simulink model "rfsoc4x2_ospfb_128"  (R2021a)
settings: Solver=VariableStepAuto  StartTime=0.0  StopTime=2048  RelTol=1e-3
undefined symbols (not defined in the file): pfb_coeff_gen_calc
libraries: xbsIndex_r4 x37092, casper_library_delays x737, casper_library_misc x68, xps_library x1
(part 117 of 339)

== system rfsoc4x2_ospfb_128/pfb_fir_real8/pol1_in2_coeffs ==
  din : Inport
  sync : Inport  Port=2
  Concat : xbsIndex_r4/Concat  num_inputs=4  dbl_ovrd=off  block_type=concat
      settings: block_version=9.1.01
  Counter : xbsIndex_r4/Counter  cnt_type=Free Running  cnt_to=Inf  operation=Up  start_count=0  cnt_by_val=1  arith_type=Unsigned  n_bits=4  bin_pt=0  load_pin=off  rst=on  en=off  explicit_period=on  period=1  use_behavioral_HDL=off  implementation=Fabric  use_rpm=on  dbl_ovrd=off  block_type=counter
      settings: xl_area=[0, 0, 0, 0, 0, 0, 0]  block_version=9.1.01
  Delay : xbsIndex_r4/Delay  rst=off  infoeditControl=Selection of Reset will increase slice count due to use of real FFs and instead of SRLs  en=off  latency=bram_latency+1+fan_latency  reg_retiming=off  dbl_ovrd=off  block_type=delay
      settings: xl_area=[0, 0, 0, 0, 0, 0, 0]  block_version=9.1.01
  Delay1 : xbsIndex_r4/Delay  rst=off  infoeditControl=Selection of Reset will increase slice count due to use of real FFs and instead of SRLs  en=off  latency=bram_latency+1+fan_latency  reg_retiming=off  dbl_ovrd=off  block_type=delay
      settings: xl_area=[0, 0, 0, 0, 0, 0, 0]  block_version=9.1.01
  ROM1 : xbsIndex_r4/ROM  depth=16  initVector=pfb_coeff_gen_calc(8, 4,'hamming',4, 1,1.3333333333333332593184650249896,1,false)  distributed_mem=Block RAM  rst=off  init_reg=0  en=off  latency=bram_latency  gui_display_data_type=Fixed-point  arith_type="Signed  (2's comp)"  n_bits=16  bin_pt=15  preci_type=Single  exp_width=8  frac_width=24  optimize=Area  use_rpm=on  dbl_ovrd=off  simulation_type=fast_sim  block_type=sprom
      settings: xl_area=[0, 0, 0, 0, 0, 0, 0]
  ROM2 : xbsIndex_r4/ROM  depth=16  initVector=pfb_coeff_gen_calc(8, 4,'hamming',4, 1,1.3333333333333332593184650249896,2,false)  distributed_mem=Block RAM  rst=off  init_reg=0  en=off  latency=bram_latency  gui_display_data_type=Fixed-point  arith_type="Signed  (2's comp)"  n_bits=16  bin_pt=15  preci_type=Single  exp_width=8  frac_width=24  optimize=Area  use_rpm=on  dbl_ovrd=off  simulation_type=fast_sim  block_type=sprom
      settings: xl_area=[0, 0, 0, 0, 0, 0, 0]
  ROM3 : xbsIndex_r4/ROM  depth=16  initVector=pfb_coeff_gen_calc(8, 4,'hamming',4, 1,1.3333333333333332593184650249896,3,false)  distributed_mem=Block RAM  rst=off  init_reg=0  en=off  latency=bram_latency  gui_display_data_type=Fixed-point  arith_type="Signed  (2's comp)"  n_bits=16  bin_pt=15  preci_type=Single  exp_width=8  frac_width=24  optimize=Area  use_rpm=on  dbl_ovrd=off  simulation_type=fast_sim  block_type=sprom
  ROM4 : xbsIndex_r4/ROM  depth=16  initVector=pfb_coeff_gen_calc(8, 4,'hamming',4, 1,1.3333333333333332593184650249896,4,false)  distributed_mem=Block RAM  rst=off  init_reg=0  en=off  latency=bram_latency  gui_display_data_type=Fixed-point  arith_type="Signed  (2's comp)"  n_bits=16  bin_pt=15  preci_type=Single  exp_width=8  frac_width=24  optimize=Area  use_rpm=on  dbl_ovrd=off  simulation_type=fast_sim  block_type=sprom
  Register : xbsIndex_r4/Register  init=0  rst=off  en=off  dbl_ovrd=off  block_type=register
      settings: xl_area=[0, 0, 0, 0, 0, 0, 0]  block_version=9.1.01
  Reinterpret{1..4} (4 alike) : xbsIndex_r4/Reinterpret  force_arith_type=on  arith_type=Unsigned  force_bin_pt=on  bin_pt=0  block_type=reinterpret
      Reinterpret1 settings: infoedit="Changes signal type without altering the binary representation.   You can changed the signal between signed and unsigned, and relocate the binary point.<P><P>Hardware notes: In hardware this block costs nothing.<P><P>Example:  Suppose the input is 6 bits wide, signed, with 2 fractional bits, and the output is forced to unsigned with 0 fractional bits.  Then an input of -2.0 (1110.00 in binary 2's complement) becomes an output of 56 (111000 in binary)."  block_version=9.1.01
      Reinterpret2 settings: infoedit="Changes signal type without altering the binary representation.   You can changed the signal between signed and unsigned, and relocate the binary point.<P><P>Hardware notes: In hardware this block costs nothing.<P><P>Example:  Suppose the input is 6 bits wide, signed, with 2 fractional bits, and the output is forced to unsigned with 0 fractional bits.  Then an input of -2.0 (1110.00 in binary 2's complement) becomes an output of 56 (111000 in binary)."  block_version=9.1.01
  fan_delay{1..4} (4 alike) : xbsIndex_r4/Delay  rst=off  infoeditControl=Selection of Reset will increase slice count due to use of real FFs and instead of SRLs  en=off  latency=fan_latency  reg_retiming=off  dbl_ovrd=off  block_type=delay
      fan_delay1 settings: block_version=11.4
      fan_delay2 settings: block_version=11.4
  dout : Outport  VectorParamsAs1DForOutWhenUnconnected=off
  sync_out : Outport  Port=2  VectorParamsAs1DForOutWhenUnconnected=off
  coeff : Outport  Port=3  VectorParamsAs1DForOutWhenUnconnected=off
  wires:
  din/1 -> Delay1/1
  Delay1/1 -> dout/1
  sync/1 -> Counter/1, Delay/1
  Delay/1 -> sync_out/1
  Concat/1 -> Register/1
  Register/1 -> coeff/1
  Counter/1 -> fan_delay1/1, fan_delay2/1, fan_delay3/1, fan_delay4/1
  fan_delay1/1 -> ROM1/1
  ROM1/1 -> Reinterpret1/1
  Reinterpret1/1 -> Concat/1
  fan_delay2/1 -> ROM2/1
  ROM2/1 -> Reinterpret2/1
  Reinterpret2/1 -> Concat/2
  fan_delay3/1 -> ROM3/1
  ROM3/1 -> Reinterpret3/1
  Reinterpret3/1 -> Concat/3
  fan_delay4/1 -> ROM4/1
  ROM4/1 -> Reinterpret4/1
  Reinterpret4/1 -> Concat/4

== system rfsoc4x2_ospfb_128/pfb_fir_real8/pol1_in2_first_tap ==
  din : Inport
  sync : Inport  Port=2
  coeffs : Inport  Port=3
  Mult : xbsIndex_r4/Mult  precision=Full  arith_type="Signed  (2's comp)"  n_bits=8  bin_pt=2  quantization=Truncate  overflow=Wrap  en=off  latency=mult_latency  use_behavioral_HDL=on  opt=Speed  use_embedded=off  optimum_pipeline=off  pipeline=on  dbl_ovrd=off  use_rpm=on  placement_style=Rectangular shape  block_type=mult
      settings: infoedit=Hardware notes: To use the internal pipeline stage of the dedicated multiplier you must select 'Pipeline for maximum performance'.  xl_area=[0, 0, 0, 0, 0, 0, 0]  block_version=9.1.01
  Reinterpret : xbsIndex_r4/Reinterpret  force_arith_type=on  arith_type="Signed  (2's comp)"  force_bin_pt=on  bin_pt=CoeffBitWidth - 1  block_type=reinterpret
      settings: infoedit="Changes signal type without altering the binary representation.   You can changed the signal between signed and unsigned, and relocate the binary point.<P><P>Hardware notes: In hardware this block costs nothing.<P><P>Example:  Suppose the input is 6 bits wide, signed, with 2 fractional bits, and the output is forced to unsigned with 0 fractional bits.  Then an input of -2.0 (1110.00 in binary 2's complement) becomes an output of 56 (111000 in binary)."  block_version=9.1.01
  Reinterpret2 : xbsIndex_r4/Reinterpret  force_arith_type=on  arith_type="Signed  (2's comp)"  force_bin_pt=on  bin_pt=BitWidthIn - 1  block_type=reinterpret
      settings: infoedit="Changes signal type without altering the binary representation.   You can changed the signal between signed and unsigned, and relocate the binary point.<P><P>Hardware notes: In hardware this block costs nothing.<P><P>Example:  Suppose the input is 6 bits wide, signed, with 2 fractional bits, and the output is forced to unsigned with 0 fractional bits.  Then an input of -2.0 (1110.00 in binary 2's complement) becomes an output of 56 (111000 in binary)."  block_version=9.1.01
  Slice : xbsIndex_r4/Slice  nbits=CoeffBitWidth  boolean_output=off  mode=Lower Bit Location + Width  bit1=0  base1=MSB of Input  bit0=0  base0=LSB of Input  dbl_ovrd=off  block_type=slice
      settings: infoedit="Extracts a given range of bits from each input sample and presents it at the output.  The output type is ordinarily unsigned with binary point at zero, but can be Boolean when the slice is one bit wide.<P><P>Hardware notes: In hardware this block costs nothing."  block_version=9.1.01
  Slice1 : xbsIndex_r4/Slice  nbits=CoeffBitWidth * (TotalTaps - 1)  boolean_output=off  mode=Two Bit Locations  bit1=0  base1=MSB of Input  bit0=CoeffBitWidth  base0=LSB of Input  dbl_ovrd=off  block_type=slice
      settings: infoedit="Extracts a given range of bits from each input sample and presents it at the output.  The output type is ordinarily unsigned with binary point at zero, but can be Boolean when the slice is one bit wide.<P><P>Hardware notes: In hardware this block costs nothing."  block_version=9.1.01
  delay_bram : casper_library_delays/delay_bram  DelayLen=2^(PFBSize-n_inputs) * n_pol_blocks  bram_latency=bram_latency  use_dsp48=off  async=off
      settings: SourceProductName=CASPER DSP Blockset
  sync_delay : casper_library_delays/sync_delay  DelayLen=2^(PFBSize-n_inputs) * n_pol_blocks
      settings: SourceProductName=CASPER DSP Blockset
  dout : Outport  VectorParamsAs1DForOutWhenUnconnected=off
  sync_out : Outport  Port=2  VectorParamsAs1DForOutWhenUnconnected=off
  coeff_out : Outport  Port=3  VectorParamsAs1DForOutWhenUnconnected=off
  taps_out : Outport  Port=4  VectorParamsAs1DForOutWhenUnconnected=off
  wires:
  coeffs/1 -> Slice1/1, Slice/1
  Reinterpret2/1 -> Mult/1
  Reinterpret/1 -> Mult/2
  Slice/1 -> Reinterpret/1
  Slice1/1 -> coeff_out/1
  sync_delay/1 -> sync_out/1
  delay_bram/1 -> dout/1
  Mult/1 -> taps_out/1
  din/1 -> Reinterpret2/1, delay_bram/1
  sync/1 -> sync_delay/1

== system rfsoc4x2_ospfb_128/pfb_fir_real8/pol1_in2_last_tap ==
  din : Inport
  sync : Inport  Port=2
  coeff : Inport  Port=3
  Delay : xbsIndex_r4/Delay  rst=off  infoeditControl=Selection of Reset will increase slice count due to use of real FFs and instead of SRLs  en=off  latency=mult_latency  reg_retiming=off  dbl_ovrd=off  block_type=delay
      settings: xl_area=[0, 0, 0, 0, 0, 0, 0]  block_version=9.1.01
  Mult : xbsIndex_r4/Mult  precision=Full  arith_type="Signed  (2's comp)"  n_bits=8  bin_pt=2  quantization=Truncate  overflow=Wrap  en=off  latency=mult_latency  use_behavioral_HDL=on  opt=Speed  use_embedded=off  optimum_pipeline=off  pipeline=on  dbl_ovrd=off  use_rpm=on  placement_style=Rectangular shape  block_type=mult
      settings: infoedit=Hardware notes: To use the internal pipeline stage of the dedicated multiplier you must select 'Pipeline for maximum performance'.  xl_area=[0, 0, 0, 0, 0, 0, 0]  block_version=9.1.01
  Reinterpret : xbsIndex_r4/Reinterpret  force_arith_type=on  arith_type="Signed  (2's comp)"  force_bin_pt=on  bin_pt=CoeffBitWidth - 1  block_type=reinterpret
      settings: infoedit="Changes signal type without altering the binary representation.   You can changed the signal between signed and unsigned, and relocate the binary point.<P><P>Hardware notes: In hardware this block costs nothing.<P><P>Example:  Suppose the input is 6 bits wide, signed, with 2 fractional bits, and the output is forced to unsigned with 0 fractional bits.  Then an input of -2.0 (1110.00 in binary 2's complement) becomes an output of 56 (111000 in binary)."  block_version=9.1.01
  Reinterpret1 : xbsIndex_r4/Reinterpret  force_arith_type=on  arith_type="Signed  (2's comp)"  force_bin_pt=on  bin_pt=BitWidthIn - 1  block_type=reinterpret
      settings: infoedit="Changes signal type without altering the binary representation.   You can changed the signal between signed and unsigned, and relocate the binary point.<P><P>Hardware notes: In hardware this block costs nothing.<P><P>Example:  Suppose the input is 6 bits wide, signed, with 2 fractional bits, and the output is forced to unsigned with 0 fractional bits.  Then an input of -2.0 (1110.00 in binary 2's complement) becomes an output of 56 (111000 in binary)."  block_version=9.1.01
  tap_out : Outport  VectorParamsAs1DForOutWhenUnconnected=off
  sync_out : Outport  Port=2  VectorParamsAs1DForOutWhenUnconnected=off
  wires:
  Delay/1 -> sync_out/1
  din/1 -> Reinterpret1/1
  sync/1 -> Delay/1
  coeff/1 -> Reinterpret/1
  Reinterpret/1 -> Mult/2
  Mult/1 -> tap_out/1
  Reinterpret1/1 -> Mult/1

== system rfsoc4x2_ospfb_128/pfb_fir_real8/pol1_in2_tap2 ==
  din : Inport
  sync : Inport  Port=2
  coeff : Inport  Port=3
  Mult : xbsIndex_r4/Mult  precision=Full  arith_type="Signed  (2's comp)"  n_bits=8  bin_pt=2  quantization=Truncate  overflow=Wrap  en=off  latency=mult_latency  use_behavioral_HDL=on  opt=Speed  use_embedded=off  optimum_pipeline=off  pipeline=on  dbl_ovrd=off  use_rpm=on  placement_style=Rectangular shape  block_type=mult
      settings: infoedit=Hardware notes: To use the internal pipeline stage of the dedicated multiplier you must select 'Pipeline for maximum performance'.  xl_area=[0, 0, 0, 0, 0, 0, 0]  block_version=9.1.01
  Reinterpret : xbsIndex_r4/Reinterpret  force_arith_type=on  arith_type="Signed  (2's comp)"  force_bin_pt=on  bin_pt=coeff_frac_width  block_type=reinterpret
      settings: infoedit="Changes signal type without altering the binary representation.   You can changed the signal between signed and unsigned, and relocate the binary point.<P><P>Hardware notes: In hardware this block costs nothing.<P><P>Example:  Suppose the input is 6 bits wide, signed, with 2 fractional bits, and the output is forced to unsigned with 0 fractional bits.  Then an input of -2.0 (1110.00 in binary 2's complement) becomes an output of 56 (111000 in binary)."  block_version=9.1.01
  Reinterpret1 : xbsIndex_r4/Reinterpret  force_arith_type=on  arith_type="Signed  (2's comp)"  force_bin_pt=on  bin_pt=data_width - 1  block_type=reinterpret
      settings: infoedit="Changes signal type without altering the binary representation.   You can changed the signal between signed and unsigned, and relocate the binary point.<P><P>Hardware notes: In hardware this block costs nothing.<P><P>Example:  Suppose the input is 6 bits wide, signed, with 2 fractional bits, and the output is forced to unsigned with 0 fractional bits.  Then an input of -2.0 (1110.00 in binary 2's complement) becomes an output of 56 (111000 in binary)."  block_version=9.1.01
  Slice : xbsIndex_r4/Slice  nbits=coeff_width  boolean_output=off  mode=Lower Bit Location + Width  bit1=0  base1=MSB of Input  bit0=0  base0=LSB of Input  dbl_ovrd=off  block_type=slice
      settings: infoedit="Extracts a given range of bits from each input sample and presents it at the output.  The output type is ordinarily unsigned with binary point at zero, but can be Boolean when the slice is one bit wide.<P><P>Hardware notes: In hardware this block costs nothing."  block_version=9.1.01
  Slice1 : xbsIndex_r4/Slice  nbits=0  boolean_output=off  mode=Two Bit Locations  bit1=0  base1=MSB of Input  bit0=coeff_width  base0=LSB of Input  dbl_ovrd=off  block_type=slice
      settings: infoedit="Extracts a given range of bits from each input sample and presents it at the output.  The output type is ordinarily unsigned with binary point at zero, but can be Boolean when the slice is one bit wide.<P><P>Hardware notes: In hardware this block costs nothing."  block_version=9.1.01
  delay_bram : casper_library_delays/delay_bram  DelayLen=delay  bram_latency=bram_latency  use_dsp48=off  async=off
      settings: SourceProductName=CASPER DSP Blockset
  sync_delay : casper_library_delays/sync_delay  DelayLen=delay
      settings: SourceProductName=CASPER DSP Blockset
  dout : Outport  VectorParamsAs1DForOutWhenUnconnected=off
  sync_out : Outport  Port=2  VectorParamsAs1DForOutWhenUnconnected=off
  coeff_out : Outport  Port=3  VectorParamsAs1DForOutWhenUnconnected=off
  taps_out : Outport  Port=4  VectorParamsAs1DForOutWhenUnconnected=off
  wires:
  delay_bram/1 -> dout/1
  din/1 -> Reinterpret1/1, delay_bram/1
  Mult/1 -> taps_out/1
  sync/1 -> sync_delay/1
  sync_delay/1 -> sync_out/1
  coeff/1 -> Slice/1, Slice1/1
  Slice1/1 -> coeff_out/1
  Slice/1 -> Reinterpret/1
  Reinterpret/1 -> Mult/2
  Reinterpret1/1 -> Mult/1

== system rfsoc4x2_ospfb_128/pfb_fir_real8/pol1_in2_tap3 ==
  din : Inport
  sync : Inport  Port=2
  coeff : Inport  Port=3
  Mult : xbsIndex_r4/Mult  precision=Full  arith_type="Signed  (2's comp)"  n_bits=8  bin_pt=2  quantization=Truncate  overflow=Wrap  en=off  latency=mult_latency  use_behavioral_HDL=on  opt=Speed  use_embedded=off  optimum_pipeline=off  pipeline=on  dbl_ovrd=off  use_rpm=on  placement_style=Rectangular shape  block_type=mult
      settings: infoedit=Hardware notes: To use the internal pipeline stage of the dedicated multiplier you must select 'Pipeline for maximum performance'.  xl_area=[0, 0, 0, 0, 0, 0, 0]  block_version=9.1.01
  Reinterpret : xbsIndex_r4/Reinterpret  force_arith_type=on  arith_type="Signed  (2's comp)"  force_bin_pt=on  bin_pt=coeff_frac_width  block_type=reinterpret
      settings: infoedit="Changes signal type without altering the binary representation.   You can changed the signal between signed and unsigned, and relocate the binary point.<P><P>Hardware notes: In hardware this block costs nothing.<P><P>Example:  Suppose the input is 6 bits wide, signed, with 2 fractional bits, and the output is forced to unsigned with 0 fractional bits.  Then an input of -2.0 (1110.00 in binary 2's complement) becomes an output of 56 (111000 in binary)."  block_version=9.1.01
  Reinterpret1 : xbsIndex_r4/Reinterpret  force_arith_type=on  arith_type="Signed  (2's comp)"  force_bin_pt=on  bin_pt=data_width - 1  block_type=reinterpret
      settings: infoedit="Changes signal type without altering the binary representation.   You can changed the signal between signed and unsigned, and relocate the binary point.<P><P>Hardware notes: In hardware this block costs nothing.<P><P>Example:  Suppose the input is 6 bits wide, signed, with 2 fractional bits, and the output is forced to unsigned with 0 fractional bits.  Then an input of -2.0 (1110.00 in binary 2's complement) becomes an output of 56 (111000 in binary)."  block_version=9.1.01
  Slice : xbsIndex_r4/Slice  nbits=coeff_width  boolean_output=off  mode=Lower Bit Location + Width  bit1=0  base1=MSB of Input  bit0=0  base0=LSB of Input  dbl_ovrd=off  block_type=slice
      settings: infoedit="Extracts a given range of bits from each input sample and presents it at the output.  The output type is ordinarily unsigned with binary point at zero, but can be Boolean when the slice is one bit wide.<P><P>Hardware notes: In hardware this block costs nothing."  block_version=9.1.01
  Slice1 : xbsIndex_r4/Slice  nbits=0  boolean_output=off  mode=Two Bit Locations  bit1=0  base1=MSB of Input  bit0=coeff_width  base0=LSB of Input  dbl_ovrd=off  block_type=slice
      settings: infoedit="Extracts a given range of bits from each input sample and presents it at the output.  The output type is ordinarily unsigned with binary point at zero, but can be Boolean when the slice is one bit wide.<P><P>Hardware notes: In hardware this block costs nothing."  block_version=9.1.01
  delay_bram : casper_library_delays/delay_bram  DelayLen=delay  bram_latency=bram_latency  use_dsp48=off  async=off
      settings: SourceProductName=CASPER DSP Blockset
  sync_delay : casper_library_delays/sync_delay  DelayLen=delay
      settings: SourceProductName=CASPER DSP Blockset
  dout : Outport  VectorParamsAs1DForOutWhenUnconnected=off
  sync_out : Outport  Port=2  VectorParamsAs1DForOutWhenUnconnected=off
  coeff_out : Outport  Port=3  VectorParamsAs1DForOutWhenUnconnected=off
  taps_out : Outport  Port=4  VectorParamsAs1DForOutWhenUnconnected=off
  wires:
  delay_bram/1 -> dout/1
  din/1 -> Reinterpret1/1, delay_bram/1
  Mult/1 -> taps_out/1
  sync/1 -> sync_delay/1
  sync_delay/1 -> sync_out/1
  coeff/1 -> Slice/1, Slice1/1
  Slice1/1 -> coeff_out/1
  Slice/1 -> Reinterpret/1
  Reinterpret/1 -> Mult/2
  Reinterpret1/1 -> Mult/1

== system rfsoc4x2_ospfb_128/pfb_fir_real8/pol1_in3_coeffs ==
  din : Inport
  sync : Inport  Port=2
  Concat : xbsIndex_r4/Concat  num_inputs=4  dbl_ovrd=off  block_type=concat
      settings: block_version=9.1.01
  Counter : xbsIndex_r4/Counter  cnt_type=Free Running  cnt_to=Inf  operation=Up  start_count=0  cnt_by_val=1  arith_type=Unsigned  n_bits=4  bin_pt=0  load_pin=off  rst=on  en=off  explicit_period=on  period=1  use_behavioral_HDL=off  implementation=Fabric  use_rpm=on  dbl_ovrd=off  block_type=counter
      settings: xl_area=[0, 0, 0, 0, 0, 0, 0]  block_version=9.1.01
  Delay : xbsIndex_r4/Delay  rst=off  infoeditControl=Selection of Reset will increase slice count due to use of real FFs and instead of SRLs  en=off  latency=bram_latency+1+fan_latency  reg_retiming=off  dbl_ovrd=off  block_type=delay
      settings: xl_area=[0, 0, 0, 0, 0, 0, 0]  block_version=9.1.01
  Delay1 : xbsIndex_r4/Delay  rst=off  infoeditControl=Selection of Reset will increase slice count due to use of real FFs and instead of SRLs  en=off  latency=bram_latency+1+fan_latency  reg_retiming=off  dbl_ovrd=off  block_type=delay
      settings: xl_area=[0, 0, 0, 0, 0, 0, 0]  block_version=9.1.01
  ROM1 : xbsIndex_r4/ROM  depth=16  initVector=pfb_coeff_gen_calc(8, 4,'hamming',4, 2,1.3333333333333332593184650249896,1,false)  distributed_mem=Block RAM  rst=off  init_reg=0  en=off  latency=bram_latency  gui_display_data_type=Fixed-point  arith_type="Signed  (2's comp)"  n_bits=16  bin_pt=15  preci_type=Single  exp_width=8  frac_width=24  optimize=Area  use_rpm=on  dbl_ovrd=off  simulation_type=fast_sim  block_type=sprom
      settings: xl_area=[0, 0, 0, 0, 0, 0, 0]
  ROM2 : xbsIndex_r4/ROM  depth=16  initVector=pfb_coeff_gen_calc(8, 4,'hamming',4, 2,1.3333333333333332593184650249896,2,false)  distributed_mem=Block RAM  rst=off  init_reg=0  en=off  latency=bram_latency  gui_display_data_type=Fixed-point  arith_type="Signed  (2's comp)"  n_bits=16  bin_pt=15  preci_type=Single  exp_width=8  frac_width=24  optimize=Area  use_rpm=on  dbl_ovrd=off  simulation_type=fast_sim  block_type=sprom
      settings: xl_area=[0, 0, 0, 0, 0, 0, 0]
  ROM3 : xbsIndex_r4/ROM  depth=16  initVector=pfb_coeff_gen_calc(8, 4,'hamming',4, 2,1.3333333333333332593184650249896,3,false)  distributed_mem=Block RAM  rst=off  init_reg=0  en=off  latency=bram_latency  gui_display_data_type=Fixed-point  arith_type="Signed  (2's comp)"  n_bits=16  bin_pt=15  preci_type=Single  exp_width=8  frac_width=24  optimize=Area  use_rpm=on  dbl_ovrd=off  simulation_type=fast_sim  block_type=sprom
      settings: xl_area=[0, 0, 0, 0, 0, 0, 0]
  ROM4 : xbsIndex_r4/ROM  depth=16  initVector=pfb_coeff_gen_calc(8, 4,'hamming',4, 2,1.3333333333333332593184650249896,4,false)  distributed_mem=Block RAM  rst=off  init_reg=0  en=off  latency=bram_latency  gui_display_data_type=Fixed-point  arith_type="Signed  (2's comp)"  n_bits=16  bin_pt=15  preci_type=Single  exp_width=8  frac_width=24  optimize=Area  use_rpm=on  dbl_ovrd=off  simulation_type=fast_sim  block_type=sprom
      settings: xl_area=[0, 0, 0, 0, 0, 0, 0]
  Register : xbsIndex_r4/Register  init=0  rst=off  en=off  dbl_ovrd=off  block_type=register
      settings: xl_area=[0, 0, 0, 0, 0, 0, 0]  block_version=9.1.01
  Reinterpret{1..4} (4 alike) : xbsIndex_r4/Reinterpret  force_arith_type=on  arith_type=Unsigned  force_bin_pt=on  bin_pt=0  block_type=reinterpret
      settings: infoedit="Changes signal type without altering the binary representation.   You can changed the signal between signed and unsigned, and relocate the binary point.<P><P>Hardware notes: In hardware this block costs nothing.<P><P>Example:  Suppose the input is 6 bits wide, signed, with 2 fractional bits, and the output is forced to unsigned with 0 fractional bits.  Then an input of -2.0 (1110.00 in binary 2's complement) becomes an output of 56 (111000 in binary)."  block_version=9.1.01
  fan_delay{1..4} (4 alike) : xbsIndex_r4/Delay  rst=off  infoeditControl=Selection of Reset will increase slice count due to use of real FFs and instead of SRLs  en=off  latency=fan_latency  reg_retiming=off  dbl_ovrd=off  block_type=delay
      settings: block_version=11.4
  dout : Outport  VectorParamsAs1DForOutWhenUnconnected=off
  sync_out : Outport  Port=2  VectorParamsAs1DForOutWhenUnconnected=off
  coeff : Outport  Port=3  VectorParamsAs1DForOutWhenUnconnected=off
  wires:
  din/1 -> Delay1/1
  Delay1/1 -> dout/1
  sync/1 -> Counter/1, Delay/1
  Delay/1 -> sync_out/1
  Concat/1 -> Register/1
  Register/1 -> coeff/1
  Counter/1 -> fan_delay1/1, fan_delay2/1, fan_delay3/1, fan_delay4/1
  fan_delay1/1 -> ROM1/1
  ROM1/1 -> Reinterpret1/1
  Reinterpret1/1 -> Concat/1
  fan_delay2/1 -> ROM2/1
  ROM2/1 -> Reinterpret2/1
  Reinterpret2/1 -> Concat/2
  fan_delay3/1 -> ROM3/1
  ROM3/1 -> Reinterpret3/1
  Reinterpret3/1 -> Concat/3
  fan_delay4/1 -> ROM4/1
  ROM4/1 -> Reinterpret4/1
  Reinterpret4/1 -> Concat/4

== system rfsoc4x2_ospfb_128/pfb_fir_real8/pol1_in3_first_tap ==
  din : Inport
  sync : Inport  Port=2
  coeffs : Inport  Port=3
  Mult : xbsIndex_r4/Mult  precision=Full  arith_type="Signed  (2's comp)"  n_bits=8  bin_pt=2  quantization=Truncate  overflow=Wrap  en=off  latency=mult_latency  use_behavioral_HDL=on  opt=Speed  use_embedded=off  optimum_pipeline=off  pipeline=on  dbl_ovrd=off  use_rpm=on  placement_style=Rectangular shape  block_type=mult
      settings: infoedit=Hardware notes: To use the internal pipeline stage of the dedicated multiplier you must select 'Pipeline for maximum performance'.  xl_area=[0, 0, 0, 0, 0, 0, 0]  block_version=9.1.01
  Reinterpret : xbsIndex_r4/Reinterpret  force_arith_type=on  arith_type="Signed  (2's comp)"  force_bin_pt=on  bin_pt=CoeffBitWidth - 1  block_type=reinterpret
      settings: infoedit="Changes signal type without altering the binary representation.   You can changed the signal between signed and unsigned, and relocate the binary point.<P><P>Hardware notes: In hardware this block costs nothing.<P><P>Example:  Suppose the input is 6 bits wide, signed, with 2 fractional bits, and the output is forced to unsigned with 0 fractional bits.  Then an input of -2.0 (1110.00 in binary 2's complement) becomes an output of 56 (111000 in binary)."  block_version=9.1.01
  Reinterpret2 : xbsIndex_r4/Reinterpret  force_arith_type=on  arith_type="Signed  (2's comp)"  force_bin_pt=on  bin_pt=BitWidthIn - 1  block_type=reinterpret
      settings: infoedit="Changes signal type without altering the binary representation.   You can changed the signal between signed and unsigned, and relocate the binary point.<P><P>Hardware notes: In hardware this block costs nothing.<P><P>Example:  Suppose the input is 6 bits wide, signed, with 2 fractional bits, and the output is forced to unsigned with 0 fractional bits.  Then an input of -2.0 (1110.00 in binary 2's complement) becomes an output of 56 (111000 in binary)."  block_version=9.1.01
  Slice : xbsIndex_r4/Slice  nbits=CoeffBitWidth  boolean_output=off  mode=Lower Bit Location + Width  bit1=0  base1=MSB of Input  bit0=0  base0=LSB of Input  dbl_ovrd=off  block_type=slice
      settings: infoedit="Extracts a given range of bits from each input sample and presents it at the output.  The output type is ordinarily unsigned with binary point at zero, but can be Boolean when the slice is one bit wide.<P><P>Hardware notes: In hardware this block costs nothing."  block_version=9.1.01
  Slice1 : xbsIndex_r4/Slice  nbits=CoeffBitWidth * (TotalTaps - 1)  boolean_output=off  mode=Two Bit Locations  bit1=0  base1=MSB of Input  bit0=CoeffBitWidth  base0=LSB of Input  dbl_ovrd=off  block_type=slice
      settings: infoedit="Extracts a given range of bits from each input sample and presents it at the output.  The output type is ordinarily unsigned with binary point at zero, but can be Boolean when the slice is one bit wide.<P><P>Hardware notes: In hardware this block costs nothing."  block_version=9.1.01
  delay_bram : casper_library_delays/delay_bram  DelayLen=2^(PFBSize-n_inputs) * n_pol_blocks  bram_latency=bram_latency  use_dsp48=off  async=off
      settings: SourceProductName=CASPER DSP Blockset
  sync_delay : casper_library_delays/sync_delay  DelayLen=2^(PFBSize-n_inputs) * n_pol_blocks
      settings: SourceProductName=CASPER DSP Blockset
  dout : Outport  VectorParamsAs1DForOutWhenUnconnected=off
  sync_out : Outport  Port=2  VectorParamsAs1DForOutWhenUnconnected=off
  coeff_out : Outport  Port=3  VectorParamsAs1DForOutWhenUnconnected=off
  taps_out : Outport  Port=4  VectorParamsAs1DForOutWhenUnconnected=off
  wires:
  coeffs/1 -> Slice1/1, Slice/1
  Reinterpret2/1 -> Mult/1
  Reinterpret/1 -> Mult/2
  Slice/1 -> Reinterpret/1
  Slice1/1 -> coeff_out/1
  sync_delay/1 -> sync_out/1
  delay_bram/1 -> dout/1
  Mult/1 -> taps_out/1
  din/1 -> Reinterpret2/1, delay_bram/1
  sync/1 -> sync_delay/1

== system rfsoc4x2_ospfb_128/pfb_fir_real8/pol1_in3_last_tap ==
  din : Inport
  sync : Inport  Port=2
  coeff : Inport  Port=3
  Delay : xbsIndex_r4/Delay  rst=off  infoeditControl=Selection of Reset will increase slice count due to use of real FFs and instead of SRLs  en=off  latency=mult_latency  reg_retiming=off  dbl_ovrd=off  block_type=delay
      settings: xl_area=[0, 0, 0, 0, 0, 0, 0]  block_version=9.1.01
  Mult : xbsIndex_r4/Mult  precision=Full  arith_type="Signed  (2's comp)"  n_bits=8  bin_pt=2  quantization=Truncate  overflow=Wrap  en=off  latency=mult_latency  use_behavioral_HDL=on  opt=Speed  use_embedded=off  optimum_pipeline=off  pipeline=on  dbl_ovrd=off  use_rpm=on  placement_style=Rectangular shape  block_type=mult
      settings: infoedit=Hardware notes: To use the internal pipeline stage of the dedicated multiplier you must select 'Pipeline for maximum performance'.  xl_area=[0, 0, 0, 0, 0, 0, 0]  block_version=9.1.01
  Reinterpret : xbsIndex_r4/Reinterpret  force_arith_type=on  arith_type="Signed  (2's comp)"  force_bin_pt=on  bin_pt=CoeffBitWidth - 1  block_type=reinterpret
      settings: infoedit="Changes signal type without altering the binary representation.   You can changed the signal between signed and unsigned, and relocate the binary point.<P><P>Hardware notes: In hardware this block costs nothing.<P><P>Example:  Suppose the input is 6 bits wide, signed, with 2 fractional bits, and the output is forced to unsigned with 0 fractional bits.  Then an input of -2.0 (1110.00 in binary 2's complement) becomes an output of 56 (111000 in binary)."  block_version=9.1.01
  Reinterpret1 : xbsIndex_r4/Reinterpret  force_arith_type=on  arith_type="Signed  (2's comp)"  force_bin_pt=on  bin_pt=BitWidthIn - 1  block_type=reinterpret
      settings: infoedit="Changes signal type without altering the binary representation.   You can changed the signal between signed and unsigned, and relocate the binary point.<P><P>Hardware notes: In hardware this block costs nothing.<P><P>Example:  Suppose the input is 6 bits wide, signed, with 2 fractional bits, and the output is forced to unsigned with 0 fractional bits.  Then an input of -2.0 (1110.00 in binary 2's complement) becomes an output of 56 (111000 in binary)."  block_version=9.1.01
  tap_out : Outport  VectorParamsAs1DForOutWhenUnconnected=off
  sync_out : Outport  Port=2  VectorParamsAs1DForOutWhenUnconnected=off
  wires:
  Delay/1 -> sync_out/1
  din/1 -> Reinterpret1/1
  sync/1 -> Delay/1
  coeff/1 -> Reinterpret/1
  Reinterpret/1 -> Mult/2
  Mult/1 -> tap_out/1
  Reinterpret1/1 -> Mult/1

== system rfsoc4x2_ospfb_128/pfb_fir_real8/pol1_in3_tap2 ==
  din : Inport
  sync : Inport  Port=2
  coeff : Inport  Port=3
  Mult : xbsIndex_r4/Mult  precision=Full  arith_type="Signed  (2's comp)"  n_bits=8  bin_pt=2  quantization=Truncate  overflow=Wrap  en=off  latency=mult_latency  use_behavioral_HDL=on  opt=Speed  use_embedded=off  optimum_pipeline=off  pipeline=on  dbl_ovrd=off  use_rpm=on  placement_style=Rectangular shape  block_type=mult
      settings: infoedit=Hardware notes: To use the internal pipeline stage of the dedicated multiplier you must select 'Pipeline for maximum performance'.  xl_area=[0, 0, 0, 0, 0, 0, 0]  block_version=9.1.01
  Reinterpret : xbsIndex_r4/Reinterpret  force_arith_type=on  arith_type="Signed  (2's comp)"  force_bin_pt=on  bin_pt=coeff_frac_width  block_type=reinterpret
      settings: infoedit="Changes signal type without altering the binary representation.   You can changed the signal between signed and unsigned, and relocate the binary point.<P><P>Hardware notes: In hardware this block costs nothing.<P><P>Example:  Suppose the input is 6 bits wide, signed, with 2 fractional bits, and the output is forced to unsigned with 0 fractional bits.  Then an input of -2.0 (1110.00 in binary 2's complement) becomes an output of 56 (111000 in binary)."  block_version=9.1.01
  Reinterpret1 : xbsIndex_r4/Reinterpret  force_arith_type=on  arith_type="Signed  (2's comp)"  force_bin_pt=on  bin_pt=data_width - 1  block_type=reinterpret
      settings: infoedit="Changes signal type without altering the binary representation.   You can changed the signal between signed and unsigned, and relocate the binary point.<P><P>Hardware notes: In hardware this block costs nothing.<P><P>Example:  Suppose the input is 6 bits wide, signed, with 2 fractional bits, and the output is forced to unsigned with 0 fractional bits.  Then an input of -2.0 (1110.00 in binary 2's complement) becomes an output of 56 (111000 in binary)."  block_version=9.1.01
  Slice : xbsIndex_r4/Slice  nbits=coeff_width  boolean_output=off  mode=Lower Bit Location + Width  bit1=0  base1=MSB of Input  bit0=0  base0=LSB of Input  dbl_ovrd=off  block_type=slice
      settings: infoedit="Extracts a given range of bits from each input sample and presents it at the output.  The output type is ordinarily unsigned with binary point at zero, but can be Boolean when the slice is one bit wide.<P><P>Hardware notes: In hardware this block costs nothing."  block_version=9.1.01
  Slice1 : xbsIndex_r4/Slice  nbits=0  boolean_output=off  mode=Two Bit Locations  bit1=0  base1=MSB of Input  bit0=coeff_width  base0=LSB of Input  dbl_ovrd=off  block_type=slice
      settings: infoedit="Extracts a given range of bits from each input sample and presents it at the output.  The output type is ordinarily unsigned with binary point at zero, but can be Boolean when the slice is one bit wide.<P><P>Hardware notes: In hardware this block costs nothing."  block_version=9.1.01
  delay_bram : casper_library_delays/delay_bram  DelayLen=delay  bram_latency=bram_latency  use_dsp48=off  async=off
      settings: SourceProductName=CASPER DSP Blockset
  sync_delay : casper_library_delays/sync_delay  DelayLen=delay
      settings: SourceProductName=CASPER DSP Blockset
  dout : Outport  VectorParamsAs1DForOutWhenUnconnected=off
  sync_out : Outport  Port=2  VectorParamsAs1DForOutWhenUnconnected=off
  coeff_out : Outport  Port=3  VectorParamsAs1DForOutWhenUnconnected=off
  taps_out : Outport  Port=4  VectorParamsAs1DForOutWhenUnconnected=off
  wires:
  delay_bram/1 -> dout/1
  din/1 -> Reinterpret1/1, delay_bram/1
  Mult/1 -> taps_out/1
  sync/1 -> sync_delay/1
  sync_delay/1 -> sync_out/1
  coeff/1 -> Slice/1, Slice1/1
  Slice1/1 -> coeff_out/1
  Slice/1 -> Reinterpret/1
  Reinterpret/1 -> Mult/2
  Reinterpret1/1 -> Mult/1

== system rfsoc4x2_ospfb_128/pfb_fir_real8/pol1_in3_tap3 ==
  din : Inport
  sync : Inport  Port=2
  coeff : Inport  Port=3
  Mult : xbsIndex_r4/Mult  precision=Full  arith_type="Signed  (2's comp)"  n_bits=8  bin_pt=2  quantization=Truncate  overflow=Wrap  en=off  latency=mult_latency  use_behavioral_HDL=on  opt=Speed  use_embedded=off  optimum_pipeline=off  pipeline=on  dbl_ovrd=off  use_rpm=on  placement_style=Rectangular shape  block_type=mult
      settings: infoedit=Hardware notes: To use the internal pipeline stage of the dedicated multiplier you must select 'Pipeline for maximum performance'.  xl_area=[0, 0, 0, 0, 0, 0, 0]  block_version=9.1.01
  Reinterpret : xbsIndex_r4/Reinterpret  force_arith_type=on  arith_type="Signed  (2's comp)"  force_bin_pt=on  bin_pt=coeff_frac_width  block_type=reinterpret
      settings: infoedit="Changes signal type without altering the binary representation.   You can changed the signal between signed and unsigned, and relocate the binary point.<P><P>Hardware notes: In hardware this block costs nothing.<P><P>Example:  Suppose the input is 6 bits wide, signed, with 2 fractional bits, and the output is forced to unsigned with 0 fractional bits.  Then an input of -2.0 (1110.00 in binary 2's complement) becomes an output of 56 (111000 in binary)."  block_version=9.1.01
  Reinterpret1 : xbsIndex_r4/Reinterpret  force_arith_type=on  arith_type="Signed  (2's comp)"  force_bin_pt=on  bin_pt=data_width - 1  block_type=reinterpret
      settings: infoedit="Changes signal type without altering the binary representation.   You can changed the signal between signed and unsigned, and relocate the binary point.<P><P>Hardware notes: In hardware this block costs nothing.<P><P>Example:  Suppose the input is 6 bits wide, signed, with 2 fractional bits, and the output is forced to unsigned with 0 fractional bits.  Then an input of -2.0 (1110.00 in binary 2's complement) becomes an output of 56 (111000 in binary)."  block_version=9.1.01
  Slice : xbsIndex_r4/Slice  nbits=coeff_width  boolean_output=off  mode=Lower Bit Location + Width  bit1=0  base1=MSB of Input  bit0=0  base0=LSB of Input  dbl_ovrd=off  block_type=slice
      settings: infoedit="Extracts a given range of bits from each input sample and presents it at the output.  The output type is ordinarily unsigned with binary point at zero, but can be Boolean when the slice is one bit wide.<P><P>Hardware notes: In hardware this block costs nothing."  block_version=9.1.01
  Slice1 : xbsIndex_r4/Slice  nbits=0  boolean_output=off  mode=Two Bit Locations  bit1=0  base1=MSB of Input  bit0=coeff_width  base0=LSB of Input  dbl_ovrd=off  block_type=slice
      settings: infoedit="Extracts a given range of bits from each input sample and presents it at the output.  The output type is ordinarily unsigned with binary point at zero, but can be Boolean when the slice is one bit wide.<P><P>Hardware notes: In hardware this block costs nothing."  block_version=9.1.01
  delay_bram : casper_library_delays/delay_bram  DelayLen=delay  bram_latency=bram_latency  use_dsp48=off  async=off
      settings: SourceProductName=CASPER DSP Blockset
  sync_delay : casper_library_delays/sync_delay  DelayLen=delay
      settings: SourceProductName=CASPER DSP Blockset
  dout : Outport  VectorParamsAs1DForOutWhenUnconnected=off
  sync_out : Outport  Port=2  VectorParamsAs1DForOutWhenUnconnected=off
  coeff_out : Outport  Port=3  VectorParamsAs1DForOutWhenUnconnected=off
  taps_out : Outport  Port=4  VectorParamsAs1DForOutWhenUnconnected=off
  wires:
  delay_bram/1 -> dout/1
  din/1 -> Reinterpret1/1, delay_bram/1
  Mult/1 -> taps_out/1
  sync/1 -> sync_delay/1
  sync_delay/1 -> sync_out/1
  coeff/1 -> Slice/1, Slice1/1
  Slice1/1 -> coeff_out/1
  Slice/1 -> Reinterpret/1
  Reinterpret/1 -> Mult/2
  Reinterpret1/1 -> Mult/1

== system rfsoc4x2_ospfb_128/pfb_fir_real8/pol1_in4_coeffs ==
  din : Inport
  sync : Inport  Port=2
  Concat : xbsIndex_r4/Concat  num_inputs=4  dbl_ovrd=off  block_type=concat
      settings: block_version=9.1.01
  Counter : xbsIndex_r4/Counter  cnt_type=Free Running  cnt_to=Inf  operation=Up  start_count=0  cnt_by_val=1  arith_type=Unsigned  n_bits=4  bin_pt=0  load_pin=off  rst=on  en=off  explicit_period=on  period=1  use_behavioral_HDL=off  implementation=Fabric  use_rpm=on  dbl_ovrd=off  block_type=counter
      settings: xl_area=[0, 0, 0, 0, 0, 0, 0]  block_version=9.1.01
  Delay : xbsIndex_r4/Delay  rst=off  infoeditControl=Selection of Reset will increase slice count due to use of real FFs and instead of SRLs  en=off  latency=bram_latency+1+fan_latency  reg_retiming=off  dbl_ovrd=off  block_type=delay
      settings: xl_area=[0, 0, 0, 0, 0, 0, 0]  block_version=9.1.01
  Delay1 : xbsIndex_r4/Delay  rst=off  infoeditControl=Selection of Reset will increase slice count due to use of real FFs and instead of SRLs  en=off  latency=bram_latency+1+fan_latency  reg_retiming=off  dbl_ovrd=off  block_type=delay
      settings: xl_area=[0, 0, 0, 0, 0, 0, 0]  block_version=9.1.01
  ROM1 : xbsIndex_r4/ROM  depth=16  initVector=pfb_coeff_gen_calc(8, 4,'hamming',4, 3,1.3333333333333332593184650249896,1,false)  distributed_mem=Block RAM  rst=off  init_reg=0  en=off  latency=bram_latency  gui_display_data_type=Fixed-point  arith_type="Signed  (2's comp)"  n_bits=16  bin_pt=15  preci_type=Single  exp_width=8  frac_width=24  optimize=Area  use_rpm=on  dbl_ovrd=off  simulation_type=fast_sim  block_type=sprom
      settings: xl_area=[0, 0, 0, 0, 0, 0, 0]
  ROM2 : xbsIndex_r4/ROM  depth=16  initVector=pfb_coeff_gen_calc(8, 4,'hamming',4, 3,1.3333333333333332593184650249896,2,false)  distributed_mem=Block RAM  rst=off  init_reg=0  en=off  latency=bram_latency  gui_display_data_type=Fixed-point  arith_type="Signed  (2's comp)"  n_bits=16  bin_pt=15  preci_type=Single  exp_width=8  frac_width=24  optimize=Area  use_rpm=on  dbl_ovrd=off  simulation_type=fast_sim  block_type=sprom
      settings: xl_area=[0, 0, 0, 0, 0, 0, 0]
  ROM3 : xbsIndex_r4/ROM  depth=16  initVector=pfb_coeff_gen_calc(8, 4,'hamming',4, 3,1.3333333333333332593184650249896,3,false)  distributed_mem=Block RAM  rst=off  init_reg=0  en=off  latency=bram_latency  gui_display_data_type=Fixed-point  arith_type="Signed  (2's comp)"  n_bits=16  bin_pt=15  preci_type=Single  exp_width=8  frac_width=24  optimize=Area  use_rpm=on  dbl_ovrd=off  simulation_type=fast_sim  block_type=sprom
      settings: xl_area=[0, 0, 0, 0, 0, 0, 0]
  ROM4 : xbsIndex_r4/ROM  depth=16  initVector=pfb_coeff_gen_calc(8, 4,'hamming',4, 3,1.3333333333333332593184650249896,4,false)  distributed_mem=Block RAM  rst=off  init_reg=0  en=off  latency=bram_latency  gui_display_data_type=Fixed-point  arith_type="Signed  (2's comp)"  n_bits=16  bin_pt=15  preci_type=Single  exp_width=8  frac_width=24  optimize=Area  use_rpm=on  dbl_ovrd=off  simulation_type=fast_sim  block_type=sprom
      settings: xl_area=[0, 0, 0, 0, 0, 0, 0]
  Register : xbsIndex_r4/Register  init=0  rst=off  en=off  dbl_ovrd=off  block_type=register
      settings: xl_area=[0, 0, 0, 0, 0, 0, 0]  block_version=9.1.01
  Reinterpret{1..4} (4 alike) : xbsIndex_r4/Reinterpret  force_arith_type=on  arith_type=Unsigned  force_bin_pt=on  bin_pt=0  block_type=reinterpret
      settings: infoedit="Changes signal type without altering the binary representation.   You can changed the signal between signed and unsigned, and relocate the binary point.<P><P>Hardware notes: In hardware this block costs nothing.<P><P>Example:  Suppose the input is 6 bits wide, signed, with 2 fractional bits, and the output is forced to unsigned with 0 fractional bits.  Then an input of -2.0 (1110.00 in binary 2's complement) becomes an output of 56 (111000 in binary)."  block_version=9.1.01
  fan_delay{1..4} (4 alike) : xbsIndex_r4/Delay  rst=off  infoeditControl=Selection of Reset will increase slice count due to use of real FFs and instead of SRLs  en=off  latency=fan_latency  reg_retiming=off  dbl_ovrd=off  block_type=delay
      settings: block_version=11.4
  dout : Outport  VectorParamsAs1DForOutWhenUnconnected=off
  sync_out : Outport  Port=2  VectorParamsAs1DForOutWhenUnconnected=off
  coeff : Outport  Port=3  VectorParamsAs1DForOutWhenUnconnected=off
  wires:
  din/1 -> Delay1/1
  Delay1/1 -> dout/1
  sync/1 -> Counter/1, Delay/1
  Delay/1 -> sync_out/1
  Concat/1 -> Register/1
  Register/1 -> coeff/1
  Counter/1 -> fan_delay1/1, fan_delay2/1, fan_delay3/1, fan_delay4/1
  fan_delay1/1 -> ROM1/1
  ROM1/1 -> Reinterpret1/1
  Reinterpret1/1 -> Concat/1
  fan_delay2/1 -> ROM2/1
  ROM2/1 -> Reinterpret2/1
  Reinterpret2/1 -> Concat/2
  fan_delay3/1 -> ROM3/1
  ROM3/1 -> Reinterpret3/1
  Reinterpret3/1 -> Concat/3
  fan_delay4/1 -> ROM4/1
  ROM4/1 -> Reinterpret4/1
  Reinterpret4/1 -> Concat/4

== system rfsoc4x2_ospfb_128/pfb_fir_real8/pol1_in4_first_tap ==
  din : Inport
  sync : Inport  Port=2
  coeffs : Inport  Port=3
  Mult : xbsIndex_r4/Mult  precision=Full  arith_type="Signed  (2's comp)"  n_bits=8  bin_pt=2  quantization=Truncate  overflow=Wrap  en=off  latency=mult_latency  use_behavioral_HDL=on  opt=Speed  use_embedded=off  optimum_pipeline=off  pipeline=on  dbl_ovrd=off  use_rpm=on  placement_style=Rectangular shape  block_type=mult
      settings: infoedit=Hardware notes: To use the internal pipeline stage of the dedicated multiplier you must select 'Pipeline for maximum performance'.  xl_area=[0, 0, 0, 0, 0, 0, 0]  block_version=9.1.01
  Reinterpret : xbsIndex_r4/Reinterpret  force_arith_type=on  arith_type="Signed  (2's comp)"  force_bin_pt=on  bin_pt=CoeffBitWidth - 1  block_type=reinterpret
      settings: infoedit="Changes signal type without altering the binary representation.   You can changed the signal between signed and unsigned, and relocate the binary point.<P><P>Hardware notes: In hardware this block costs nothing.<P><P>Example:  Suppose the input is 6 bits wide, signed, with 2 fractional bits, and the output is forced to unsigned with 0 fractional bits.  Then an input of -2.0 (1110.00 in binary 2's complement) becomes an output of 56 (111000 in binary)."  block_version=9.1.01
  Reinterpret2 : xbsIndex_r4/Reinterpret  force_arith_type=on  arith_type="Signed  (2's comp)"  force_bin_pt=on  bin_pt=BitWidthIn - 1  block_type=reinterpret
      settings: infoedit="Changes signal type without altering the binary representation.   You can changed the signal between signed and unsigned, and relocate the binary point.<P><P>Hardware notes: In hardware this block costs nothing.<P><P>Example:  Suppose the input is 6 bits wide, signed, with 2 fractional bits, and the output is forced to unsigned with 0 fractional bits.  Then an input of -2.0 (1110.00 in binary 2's complement) becomes an output of 56 (111000 in binary)."  block_version=9.1.01
  Slice : xbsIndex_r4/Slice  nbits=CoeffBitWidth  boolean_output=off  mode=Lower Bit Location + Width  bit1=0  base1=MSB of Input  bit0=0  base0=LSB of Input  dbl_ovrd=off  block_type=slice
      settings: infoedit="Extracts a given range of bits from each input sample and presents it at the output.  The output type is ordinarily unsigned with binary point at zero, but can be Boolean when the slice is one bit wide.<P><P>Hardware notes: In hardware this block costs nothing."  block_version=9.1.01
  Slice1 : xbsIndex_r4/Slice  nbits=CoeffBitWidth * (TotalTaps - 1)  boolean_output=off  mode=Two Bit Locations  bit1=0  base1=MSB of Input  bit0=CoeffBitWidth  base0=LSB of Input  dbl_ovrd=off  block_type=slice
      settings: infoedit="Extracts a given range of bits from each input sample and presents it at the output.  The output type is ordinarily unsigned with binary point at zero, but can be Boolean when the slice is one bit wide.<P><P>Hardware notes: In hardware this block costs nothing."  block_version=9.1.01
  delay_bram : casper_library_delays/delay_bram  DelayLen=2^(PFBSize-n_inputs) * n_pol_blocks  bram_latency=bram_latency  use_dsp48=off  async=off
      settings: SourceProductName=CASPER DSP Blockset
  sync_delay : casper_library_delays/sync_delay  DelayLen=2^(PFBSize-n_inputs) * n_pol_blocks
      settings: SourceProductName=CASPER DSP Blockset
  dout : Outport  VectorParamsAs1DForOutWhenUnconnected=off
  sync_out : Outport  Port=2  VectorParamsAs1DForOutWhenUnconnected=off
  coeff_out : Outport  Port=3  VectorParamsAs1DForOutWhenUnconnected=off
  taps_out : Outport  Port=4  VectorParamsAs1DForOutWhenUnconnected=off
  wires:
  coeffs/1 -> Slice1/1, Slice/1
  Reinterpret2/1 -> Mult/1
  Reinterpret/1 -> Mult/2
  Slice/1 -> Reinterpret/1
  Slice1/1 -> coeff_out/1
  sync_delay/1 -> sync_out/1
  delay_bram/1 -> dout/1
  Mult/1 -> taps_out/1
  din/1 -> Reinterpret2/1, delay_bram/1
  sync/1 -> sync_delay/1
